simulink subsystem "Dynamics"  (R2024b)
settings: Solver=VariableStepAuto  StartTime=0.0  StopTime=10.0  RelTol=1e-3
settings Model: Creator=marco  LastModifiedBy=domac

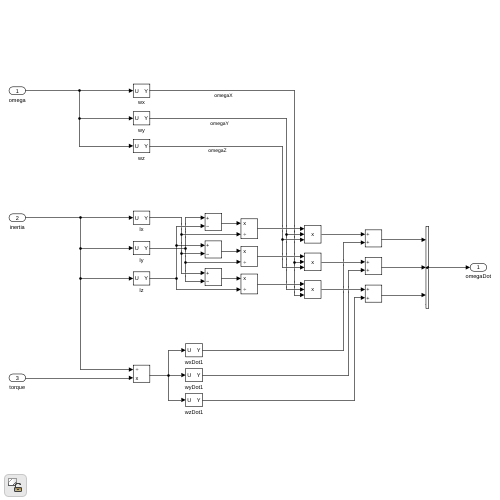
[thumbnail: Simulink's stored preview of the top-level diagram]
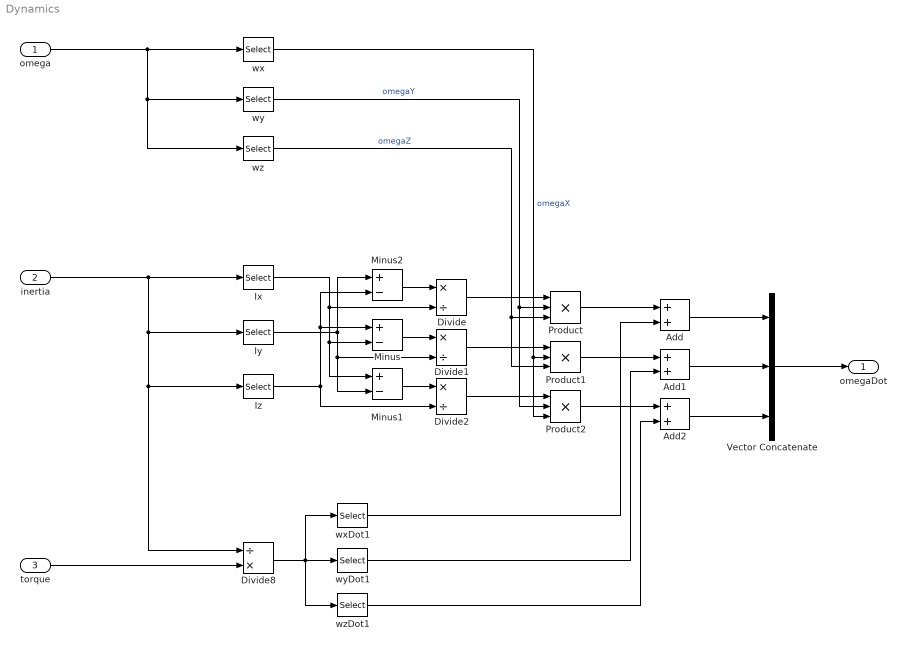
== system Dynamics ==
  omega : Inport
  inertia : Inport  Port=2
  torque : Inport  Port=3
  Add : Sum
  Add1 : Sum
  Add2 : Sum
  Divide : Product  Inputs=*/
  Divide1 : Product  Inputs=*/
  Divide2 : Product  Inputs=*/
  Divide8 : Product  Inputs=/*
  Ix : Selector  NumberOfDimensions=2  InputPortWidth=3  IndexOptions=Index vector (dialog),Select all  Indices=1,1  OutputSizes=1,1
  Iy : Selector  NumberOfDimensions=2  InputPortWidth=3  IndexOptions=Index vector (dialog),Select all  Indices=2,1  OutputSizes=1,1
  Iz : Selector  NumberOfDimensions=2  InputPortWidth=3  IndexOptions=Index vector (dialog),Select all  Indices=3,1  OutputSizes=1,1
  Minus : Sum  Inputs=+-
  Minus1 : Sum  Inputs=+-
  Minus2 : Sum  Inputs=+-
  Product : Product  Inputs=3
  Product1 : Product  Inputs=3
  Product2 : Product  Inputs=3
  Vector Concatenate : Concatenate  NumInputs=3  Mode=Multidimensional array
  wx : Selector  NumberOfDimensions=2  InputPortWidth=3  IndexOptions=Index vector (dialog),Select all  Indices=1,1  OutputSizes=1,1
  wxDot1 : Selector  NumberOfDimensions=2  InputPortWidth=3  IndexOptions=Index vector (dialog),Select all  Indices=1,1  OutputSizes=1,1
  wy : Selector  NumberOfDimensions=2  InputPortWidth=3  IndexOptions=Index vector (dialog),Select all  Indices=2,1  OutputSizes=1,1
  wyDot1 : Selector  NumberOfDimensions=2  InputPortWidth=3  IndexOptions=Index vector (dialog),Select all  Indices=2,1  OutputSizes=1,1
  wz : Selector  NumberOfDimensions=2  InputPortWidth=3  IndexOptions=Index vector (dialog),Select all  Indices=3,1  OutputSizes=1,1
  wzDot1 : Selector  NumberOfDimensions=2  InputPortWidth=3  IndexOptions=Index vector (dialog),Select all  Indices=3,1  OutputSizes=1,1
  omegaDot : Outport
  wires:
  Product1/1 -> Add1/1
  Iz/1 -> Divide2/2, Minus2/2, Minus/1
  Iy/1 -> Minus2/1, Divide1/2, Minus1/2
  Minus2/1 -> Divide/1
  Minus/1 -> Divide1/1
  Minus1/1 -> Divide2/1
  Ix/1 -> Divide/2, Minus/2, Minus1/1
  Divide1/1 -> Product1/1
  wx/1 -> Product1/2, Product2/3  "omegaX"
  Vector Concatenate/1 -> omegaDot/1
  Divide2/1 -> Product2/1
  wy/1 -> Product/2, Product2/2  "omegaY"
  Divide/1 -> Product/1
  wz/1 -> Product/3, Product1/3  "omegaZ"
  Product/1 -> Add/1
  omega/1 -> wx/1, wy/1, wz/1
  inertia/1 -> Ix/1, Iy/1, Iz/1, Divide8/1
  Product2/1 -> Add2/1
  torque/1 -> Divide8/2
  Divide8/1 -> wyDot1/1, wxDot1/1, wzDot1/1
  wxDot1/1 -> Add/2
  wyDot1/1 -> Add1/2
  wzDot1/1 -> Add2/2
  Add/1 -> Vector Concatenate/1
  Add1/1 -> Vector Concatenate/2
  Add2/1 -> Vector Concatenate/3
